simulink model "Pipeline_System_Model"  (R2025b)
settings: Solver=VariableStepAuto  StartTime=0.0  StopTime=0.5  RelTol=1e-3
libraries: simulink x1
settings Model: Creator=Gowtham  LastModifiedBy=Gowtham

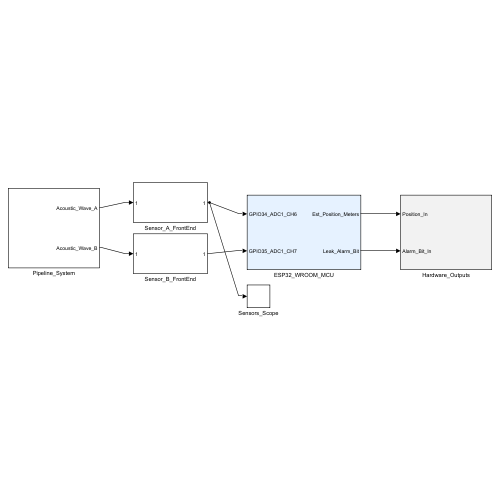
[thumbnail: Simulink's stored preview of the top-level diagram]
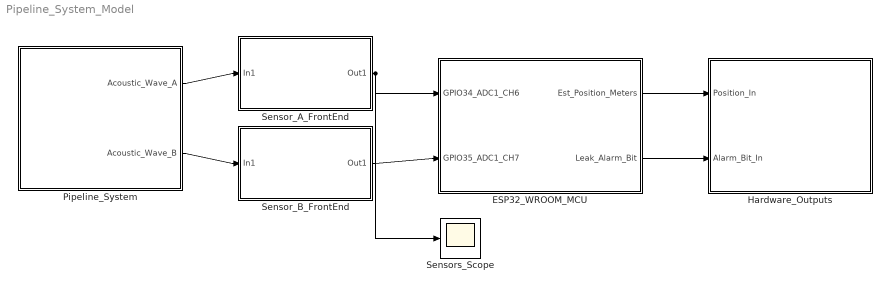
== system Pipeline_System_Model ==
  ESP32_WROOM_MCU : Subsystem
  Hardware_Outputs : Subsystem
  Pipeline_System : Subsystem
  Sensor_A_FrontEnd : Subsystem
  Sensor_B_FrontEnd : Subsystem
  Sensors_Scope : Scope
  wires:
  Pipeline_System/1(Acoustic_Wave_A) -> Sensor_A_FrontEnd/1(In1)
  Pipeline_System/2(Acoustic_Wave_B) -> Sensor_B_FrontEnd/1(In1)
  Sensor_A_FrontEnd/1(Out1) -> ESP32_WROOM_MCU/1(GPIO34_ADC1_CH6), Sensors_Scope/1
  Sensor_B_FrontEnd/1(Out1) -> ESP32_WROOM_MCU/2(GPIO35_ADC1_CH7)
  ESP32_WROOM_MCU/1(Est_Position_Meters) -> Hardware_Outputs/1(Position_In)
  ESP32_WROOM_MCU/2(Leak_Alarm_Bit) -> Hardware_Outputs/2(Alarm_Bit_In)

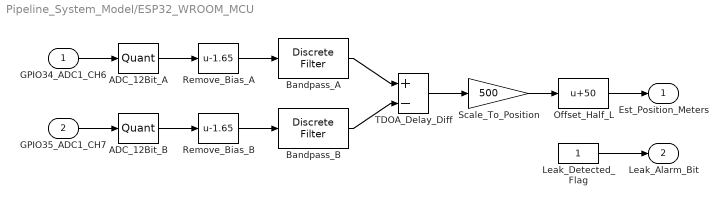
== system Pipeline_System_Model/ESP32_WROOM_MCU ==
  GPIO34_ADC1_CH6 : Inport
  GPIO35_ADC1_CH7 : Inport  Port=2
  ADC_12Bit_A : Quantizer  QuantizationInterval=3.3/4095
  ADC_12Bit_B : Quantizer  QuantizationInterval=3.3/4095
  Bandpass_A : DiscreteFilter
  Bandpass_B : DiscreteFilter
  Leak_Detected_Flag : Constant
  Offset_Half_L : Bias  Bias=50  SaturateOnIntegerOverflow=off
  Remove_Bias_A : Bias  Bias=-1.65  SaturateOnIntegerOverflow=off
  Remove_Bias_B : Bias  Bias=-1.65  SaturateOnIntegerOverflow=off
  Scale_To_Position : Gain  Gain=500
  TDOA_Delay_Diff : Sum  Inputs=+-
  Est_Position_Meters : Outport
  Leak_Alarm_Bit : Outport  Port=2
  wires:
  GPIO34_ADC1_CH6/1 -> ADC_12Bit_A/1
  GPIO35_ADC1_CH7/1 -> ADC_12Bit_B/1
  ADC_12Bit_A/1 -> Remove_Bias_A/1
  ADC_12Bit_B/1 -> Remove_Bias_B/1
  Remove_Bias_A/1 -> Bandpass_A/1
  Remove_Bias_B/1 -> Bandpass_B/1
  Bandpass_A/1 -> TDOA_Delay_Diff/1
  Bandpass_B/1 -> TDOA_Delay_Diff/2
  TDOA_Delay_Diff/1 -> Scale_To_Position/1
  Scale_To_Position/1 -> Offset_Half_L/1
  Offset_Half_L/1 -> Est_Position_Meters/1
  Leak_Detected_Flag/1 -> Leak_Alarm_Bit/1

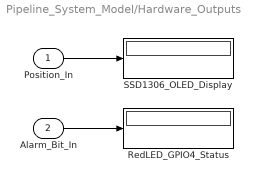
== system Pipeline_System_Model/Hardware_Outputs ==
  Position_In : Inport
  Alarm_Bit_In : Inport  Port=2
  RedLED_GPIO4_Status : Display
  SSD1306_OLED_Display : Display
  wires:
  Position_In/1 -> SSD1306_OLED_Display/1
  Alarm_Bit_In/1 -> RedLED_GPIO4_Status/1

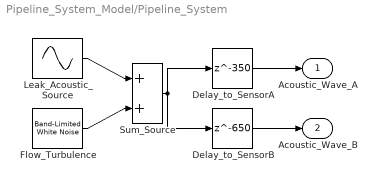
== system Pipeline_System_Model/Pipeline_System ==
  Delay_to_SensorA : Delay  DelayLength=350
  Delay_to_SensorB : Delay  DelayLength=650
  Flow_Turbulence : simulink/Sources/Band-Limited White Noise  Cov=0.001  Ts=0.0001  seed=[23341]
  Leak_Acoustic_Source : Sin  Amplitude=0.5  Frequency=2*pi*850  SampleTime=0
  Sum_Source : Sum
  Acoustic_Wave_A : Outport
  Acoustic_Wave_B : Outport  Port=2
  wires:
  Leak_Acoustic_Source/1 -> Sum_Source/1
  Flow_Turbulence/1 -> Sum_Source/2
  Sum_Source/1 -> Delay_to_SensorA/1, Delay_to_SensorB/1
  Delay_to_SensorA/1 -> Acoustic_Wave_A/1
  Delay_to_SensorB/1 -> Acoustic_Wave_B/1

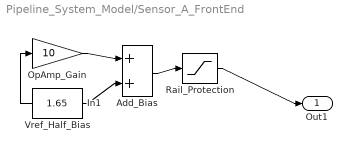
== system Pipeline_System_Model/Sensor_A_FrontEnd ==
  In1 : Inport
  Add_Bias : Sum
  OpAmp_Gain : Gain  Gain=10
  Rail_Protection : Saturate  UpperLimit=3.3  LowerLimit=0.0
  Vref_Half_Bias : Constant  Value=1.65
  Out1 : Outport
  wires:
  In1/1 -> OpAmp_Gain/1
  OpAmp_Gain/1 -> Add_Bias/1
  Vref_Half_Bias/1 -> Add_Bias/2
  Add_Bias/1 -> Rail_Protection/1
  Rail_Protection/1 -> Out1/1

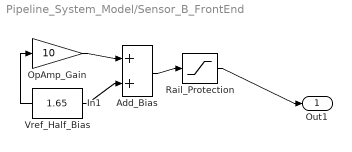
== system Pipeline_System_Model/Sensor_B_FrontEnd ==
  In1 : Inport
  Add_Bias : Sum
  OpAmp_Gain : Gain  Gain=10
  Rail_Protection : Saturate  UpperLimit=3.3  LowerLimit=0.0
  Vref_Half_Bias : Constant  Value=1.65
  Out1 : Outport
  wires:
  In1/1 -> OpAmp_Gain/1
  OpAmp_Gain/1 -> Add_Bias/1
  Vref_Half_Bias/1 -> Add_Bias/2
  Add_Bias/1 -> Rail_Protection/1
  Rail_Protection/1 -> Out1/1
